simulink model "project"  (R2025a)
settings: Solver=VariableStepAuto  StartTime=0.0  StopTime=0.5  RelTol=1e-3
libraries: spsSeriesRLCBranchLib x7, spsMosfetLib x4, spsVoltageMeasurementLib x3, slpidlib x2, simulink x2, spsCurrentMeasurementLib x2, spsFirstOrderFilterLib x2, spsACVoltageSourceLib x1, spsDiodeLib x1, spsIGBTLib x1, spsPLLLib x1, spsPVArrayLib x1
settings Model: Creator=RYAN CHAN  LastModifiedBy=sharv
settings DebuggingCC: UnconnectedInputMsg=warning  UnconnectedOutputMsg=warning  UnconnectedLineMsg=warning
settings ModelReferenceCC: EnableRefExpFcnMdlSchedulingChecks=on
settings RTWCC: GPUComputeCapability=3.5  DLArmComputeVersion=19.05

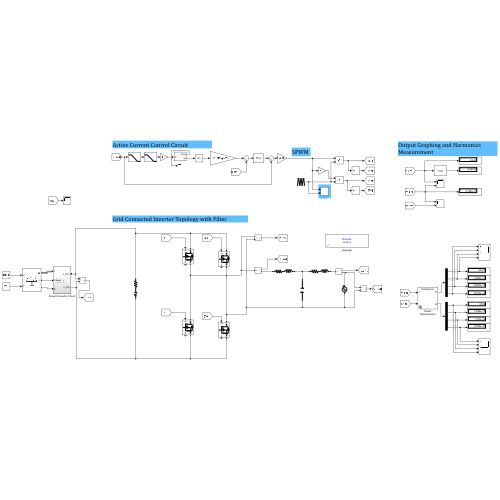
[thumbnail: Simulink's stored preview of the top-level diagram]
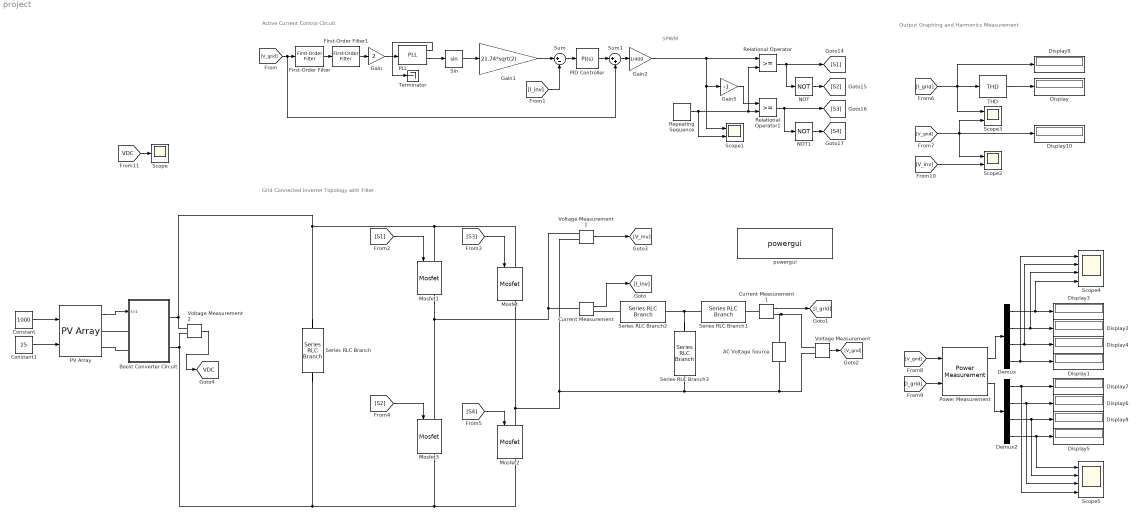
== system project ==
  note: Active Current Control Circuit
  note: Grid Connected Inverter Topology with Filter
  note: SPWM
  note: Output Graphing and Harmonics Measurement
  AC Voltage Source : spsACVoltageSourceLib/AC Voltage Source  Amplitude=230*sqrt(2)  Phase=0  Frequency=50  SampleTime=0  Measurements=None  BusType=swing  Pref=10e3  Qref=0  Qmin=-inf  Qmax=+inf
  Boost Converter Circuit : Subsystem
  Constant : Constant  Value=1000
  Constant1 : Constant  Value=25
  Current Measurement : spsCurrentMeasurementLib/Current Measurement  PhasorSimulation=off  OutputType=Complex  PSBequivalent=0
  Current Measurement1 : spsCurrentMeasurementLib/Current Measurement  PhasorSimulation=off  OutputType=Complex  PSBequivalent=0
  Demux : Demux
  Demux2 : Demux
  Display{,1..10} (11 alike) : Display
  First-Order Filter : spsFirstOrderFilterLib/First-Order Filter  FilterType=Lowpass  Tc=1/(2*pi*50)  Ts=0  Initialize=off  Vac_Init=[0, 0, 60]  Vdc_Init=0  PlotResponse=off  FreqRange="[0,  200,  1]"
  First-Order Filter1 : spsFirstOrderFilterLib/First-Order Filter  FilterType=Lowpass  Tc=1/(2*pi*50)  Ts=0  Initialize=off  Vac_Init=[0, 0, 60]  Vdc_Init=0  PlotResponse=off  FreqRange="[0,  200,  1]"
  Gain : Gain  Gain=2
  Gain1 : Gain  Gain=21.74*sqrt(2)
  Gain2 : Gain  Gain=1/400
  Gain5 : Gain  Gain=-1
  Mosfet{,1..3} (4 alike) : spsMosfetLib/Mosfet  Ron=0.1  Lon=0  Rd=0.01  Vfd=0  IC=0  Rs=1e5  Cs=inf  Measurements=on
  NOT : Logic  Operator=NOT  AllPortsSameDT=off  OutDataTypeStr=boolean
  NOT1 : Logic  Operator=NOT  AllPortsSameDT=off  OutDataTypeStr=boolean
  PID Controller : slpidlib/PID Controller  Controller=PI  Form=Parallel  TimeDomain=Continuous-time  UseExternalTs=off  SampleTime=-1  IntegratorMethod=Forward Euler  FilterMethod=Forward Euler  ControllerParametersSource=internal  P=10.06  I=0.1509  UseKiTs=off  D=0  UseExternalDerivativeSource=off  N=100  UseFilter=on  TunerSelectOption=Transfer Function Based (PID Tuner App)  InitialConditionSource=internal  InitialConditionForIntegrator=0  InitialConditionForFilter=0  DifferentiatorICPrevScaledInput=0  ExternalReset=none  TrackingMode=off  Kt=1  LimitOutput=off  SatLimitsSource=internal  UpperSaturationLimit=inf  LowerSaturationLimit=-inf  LinearizeAsGain=on  AntiWindupMode=none  Kb=1  LimitIntegrator=off  UpperIntegratorSaturationLimit=inf  LowerIntegratorSaturationLimit=-inf  POutMin=[]  POutMax=[]  IOutMin=[]  IOutMax=[]  DOutMin=[]  DOutMax=[]  NOutMin=[]  NOutMax=[]  SumOutMin=[]  SumOutMax=[]  SaturationOutMin=[]  SaturationOutMax=[]  PParamMin=[]  PParamMax=[]  IParamMin=[]  IParamMax=[]  DParamMin=[]  DParamMax=[]  NParamMin=[]  NParamMax=[]  KbParamMin=[]  KbParamMax=[]  KtParamMin=[]  KtParamMax=[]  KbOutMin=[]  KbOutMax=[]  KtOutMin=[]  KtOutMax=[]  IntegratorOutMin=[]  IntegratorOutMax=[]  FilterOutMin=[]  FilterOutMax=[]  SumI1OutMin=[]  SumI1OutMax=[]  SumI2OutMin=[]  SumI2OutMax=[]  SumI3OutMin=[]  SumI3OutMax=[]  SumI4OutMin=[]  SumI4OutMax=[]  SumDOutMin=[]  SumDOutMax=[]  DifferentiatorOutMin=[]  DifferentiatorOutMax=[]  FilterDiffOutCoefMin=[]  FilterDiffOutCoefMax=[]  ReciprocalOutMin=[]  ReciprocalOutMax=[]  SumDenOutMin=[]  SumDenOutMax=[]  SumNumOutMin=[]  SumNumOutMax=[]  DivideOutMin=[]  DivideOutMax=[]  UdiffTsProdOutMin=[]  UdiffTsProdOutMax=[]  NTsProdOutMin=[]  NTsProdOutMax=[]  UintegralTsProdOutMin=[]  UintegralTsProdOutMax=[]  UngainTsProdOutMin=[]  UngainTsProdOutMax=[]  ClampingZeroOutDataTypeStr=Inherit: Inherit via back propagation  ClampingZeroOutMin=[]  ClampingZeroOutMax=[]  FilterDenConstantOutDataTypeStr=Inherit: Inherit via back propagation  FilterDenConstantOutMin=[]  FilterDenConstantOutMax=[]  PCopyOutDataTypeStr=Inherit: Inherit via back propagation  PCopyOutMin=[]  PCopyOutMax=[]  NCopyOutDataTypeStr=Inherit: Inherit via back propagation  NCopyOutMin=[]  NCopyOutMax=[]  IntegratorContinuousStateAttributes=''  IntegratorStateMustResolveToSignalObject=off  IntegratorRTWStateStorageClass=Auto  FilterContinuousStateAttributes=''  FilterStateMustResolveToSignalObject=off  FilterRTWStateStorageClass=Auto  ParallelPVariant=InternalParameters  IdealPVariant=Disabled  IVariant=InternalParameters  DVariant=Disabled  IntegratorVariant=Continuous  SatVariant=Disabled  AWVariant=Passthrough  PCopyVariant=Disabled  TRVariant=Disabled  FdbkBlocksVariant=Forward  IdealPFdbkVariant=Disabled  SatFdbkVariant=Disabled  DerivativeFilterVariant=Disabled  NVariant=Disabled  NCopyVariant=Disabled_SignalSpec  FilterICVariant=Disabled  IntegratorICVariant=InternalICs  ExternalResetVariant=Disabled  TRSumVariant=Passthrough  SumFdbkVariant=Disabled  SumVariant=Sum_PI  TsampFilterVariant=InternalTs  TsampNgainVariant=Passthrough  TsampIntegralVariant=Disabled_SignalSpec  ExternalSaturationOutDataTypeStr=Inherit: Same as second input  DerivativeSourceVariant=Disabled  PreIntVariant=InternalPreInt
  PLL : spsPLLLib/PLL  Fmin=45  Par_Init=[0, 50]  ParK=[180, 3200, 1]  TcD=162e-6  MaxRateChangeFreq=12  FilterCutOffFreq=25  Ts=0  AGC=on
  PV Array : spsPVArrayLib/PV Array  Npar=47  Nser=10  PlotType=array @ 25 deg.C & specified irradiances  S_vec="[ 1000  500  100 ]"  Temp_C_vec="[ 45 25  ]"  ModuleName=User-defined  PlotWhenSelected=off  Pm=213.15  Ncell=60  Voc=36.3  Isc=7.84  Vm=29  Im=7.35  beta_Voc_pc=-0.36099  alpha_Isc_pc=0.102  beta_Voc=-0.13104  alpha_Isc=0.0079968  IL=7.8654  I0=2.9273e-10  nI=0.98119  Rsh=313.0553  Rs=0.39381  RobustModel=off  RobustCellTemperature=313.3991  BAL=on  Tc=1e-6  Tfilter=5e-5
  Power Measurement : eePowerMeasurement/Power Measurement  LabelModeActiveChoice=Continuous  F=50  K=[1 3 5 7]  Ts=0
  Relational Operator : RelationalOperator  OutDataTypeStr=boolean  RndMeth=Simplest  InputSameDT=off
  Relational Operator1 : RelationalOperator  OutDataTypeStr=boolean  RndMeth=Simplest  InputSameDT=off
  Repeating Sequence : simulink/Sources/Repeating Sequence  rep_seq_t=[0 1e-5 2e-5]  rep_seq_y=[-1 1 -1]
  Scope : Scope
      settings: DataLoggingVariableName=ScopeData4
  Scope1 : Scope  NumInputPorts=2
      settings: ActiveDisplayYMinimum=-1.1382  ActiveDisplayYMaximum=0.98886
  Scope2 : Scope  NumInputPorts=2
      settings: ActiveDisplayYMinimum=-406.58639918226481  ActiveDisplayYMaximum=406.58639918226481  DataLoggingVariableName=ScopeData3
  Scope3 : Scope  NumInputPorts=2
      settings: ActiveDisplayYMinimum=-43.30712  ActiveDisplayYMaximum=44.57517  DataLoggingVariableName=ScopeData2
  Scope4 : Scope  NumInputPorts=4
      settings: ActiveDisplayYMinimum=-27.85377883509021  ActiveDisplayYMaximum=31.806771928915644
  Scope5 : Scope  NumInputPorts=4
      settings: ActiveDisplayYMinimum=-12.72391  ActiveDisplayYMaximum=12.80046  DataLoggingVariableName=ScopeData2
  Series RLC Branch : spsSeriesRLCBranchLib/Series RLC Branch  LConnTagsString=__new0  RConnTagsString=__new0  BranchType=RC  Resistance=32  Inductance=1e-3  SetiL0=off  InitialCurrent=0  Capacitance=1e-6  Setx0=off  InitialVoltage=0  Measurements=None
  Series RLC Branch1 : spsSeriesRLCBranchLib/Series RLC Branch  LConnTagsString=__new0  RConnTagsString=__new0  BranchType=RL  Resistance=15e-3  Inductance=1.74e-3  SetiL0=off  InitialCurrent=0  Capacitance=1e-6  Setx0=off  InitialVoltage=0  Measurements=None
  Series RLC Branch2 : spsSeriesRLCBranchLib/Series RLC Branch  LConnTagsString=__new0  RConnTagsString=__new0  BranchType=RL  Resistance=15e-3  Inductance=1.63e-3  SetiL0=off  InitialCurrent=0  Capacitance=1e-6  Setx0=off  InitialVoltage=0  Measurements=None
  Series RLC Branch3 : spsSeriesRLCBranchLib/Series RLC Branch  LConnTagsString=__new0  RConnTagsString=__new0  BranchType=C  Resistance=1e-3  Inductance=1e-3  SetiL0=off  InitialCurrent=0  Capacitance=15e-6  Setx0=off  InitialVoltage=0  Measurements=None
  Sin : Trigonometry
  Sum : Sum  Inputs=|+-
  Sum1 : Sum  Inputs=|++
  THD : spsTHDLib/THD  Freq=50  Ts=0
  Terminator : Terminator
  Voltage Measurement : spsVoltageMeasurementLib/Voltage Measurement  PhasorSimulation=off  OutputType=Complex  PSBequivalent=0
  Voltage Measurement1 : spsVoltageMeasurementLib/Voltage Measurement  PhasorSimulation=off  OutputType=Complex  PSBequivalent=0
  Voltage Measurement2 : spsVoltageMeasurementLib/Voltage Measurement  PhasorSimulation=off  OutputType=Complex  PSBequivalent=0
  powergui : spspowerguiLib/powergui  Priority=1  SimulationMode=Discrete  SampleTime=1e-6  frequency=60  Iterations=50  frequencyindice=50  Pbase=100e6  ErrMax=1e-4  UnitsV=kV  UnitsW=MW  buscounter=0  FunctionMessages=off  echomessages=off  EnableUseOfTLC=off  CurrentSourceSwitches=off  DisableSnubberDevices=off  DisableRonSwitches=off  DisableVfSwitches=off  DisplayEquations=off  AutomaticDiscreteSolvers=off  SolverType=Tustin/Backward Euler (TBE)  Interpol=off  ExternalGateDelay=off  methode=off  Ts=100  x0status=blocks  SPID=on  SwTol=0  HookPort=off  NonlinearTolerance=1e-4  nMaxIteration=100  ContinueOnMaxIteration=off  RestoreLinks=warning  ResistiveCurrentMeasurement=off  Frange=[0:2:500]  Ylog=off  Xlog=on  ShowGrid=off  save=off  variable=ZData  structure=0  ZoomFFT=off  StartTime=0.0  cycles=1  DisplayStyle=1  fundamental=60  FreqAxis=off  MaxFrequency=1000  frequencyindicesteady=1  RmsSteady=1  display=off
  tag scope: VDC=global
  wires:
  [V_grid] -> Sum1/2, First-Order Filter/1
  First-Order Filter/1 -> First-Order Filter1/1
  First-Order Filter1/1 -> Gain/1
  Sin/1 -> Gain1/1
  Gain1/1 -> Sum/1
  Sum/1 -> PID Controller/1
  [I_inv] -> Sum/2
  PID Controller/1 -> Sum1/1
  Sum1/1 -> Gain2/1
  Gain2/1 -> Relational Operator/1, Scope1/1, Gain5/1
  Relational Operator1/1 -> NOT1/1, [S3]
  NOT1/1 -> [S4]
  NOT/1 -> [S2]
  Gain5/1 -> Relational Operator1/1
  Repeating Sequence/1 -> Scope1/2, Relational Operator1/2, Relational Operator/2
  Relational Operator/1 -> NOT/1, [S1]
  Current Measurement1/1 -> [I_grid]
  [S3] -> Mosfet/1
  Current Measurement/1 -> [I_inv]
  [S1] -> Mosfet1/1
  Voltage Measurement/1 -> [V_grid]
  [S2] -> Mosfet3/1
  [S4] -> Mosfet2/1
  Gain/1 -> PLL/1
  PLL/2 -> Sin/1
  PLL/1 -> Terminator/1
  [I_grid] -> Display9/1, THD/1, Scope3/1
  [V_grid] -> Scope2/1, Display10/1, Scope3/2
  THD/1 -> Display/1
  [I_grid] -> Power Measurement/2
  [V_grid] -> Power Measurement/1
  Power Measurement/1 -> Demux/1
  Demux/3 -> Scope4/2, Display4/1
  Demux/1 -> Scope4/4, Display3/1
  Demux/4 -> Display1/1, Scope4/1
  Demux/2 -> Scope4/3, Display2/1
  Demux2/2 -> Scope5/3, Display6/1
  Demux2/4 -> Scope5/1, Display5/1
  Demux2/1 -> Scope5/4, Display7/1
  Demux2/3 -> Display8/1, Scope5/2
  Power Measurement/2 -> Demux2/1
  Voltage Measurement1/1 -> [V_inv]
  [V_inv] -> Scope2/2
  PV Array/1 -> Boost Converter Circuit/1(In1)
  Constant1/1 -> PV Array/2
  Voltage Measurement2/1 -> [VDC]
  Constant/1 -> PV Array/1
  [VDC] -> Scope/1
  connections:
  Voltage Measurement/LConn2 -- AC Voltage Source/LConn1 -- Series RLC Branch3/RConn1 -- Voltage Measurement1/LConn2 -- Mosfet2/LConn1 -- Mosfet/RConn1
  Voltage Measurement/LConn1 -- Current Measurement1/RConn1 -- AC Voltage Source/RConn1
  Boost Converter Circuit/RConn2 -- Mosfet2/RConn1 -- Mosfet3/RConn1 -- Series RLC Branch/RConn1 -- Voltage Measurement2/LConn2
  Current Measurement/LConn1 -- Voltage Measurement1/LConn1 -- Mosfet3/LConn1 -- Mosfet1/RConn1
  Boost Converter Circuit/RConn1 -- Voltage Measurement2/LConn1 -- Mosfet1/LConn1 -- Mosfet/LConn1 -- Series RLC Branch/LConn1
  Series RLC Branch2/RConn1 -- Series RLC Branch1/LConn1 -- Series RLC Branch3/LConn1
  Current Measurement1/LConn1 -- Series RLC Branch1/RConn1
  Series RLC Branch2/LConn1 -- Current Measurement/RConn1
  Boost Converter Circuit/LConn1 -- PV Array/RConn1
  Boost Converter Circuit/LConn2 -- PV Array/RConn2

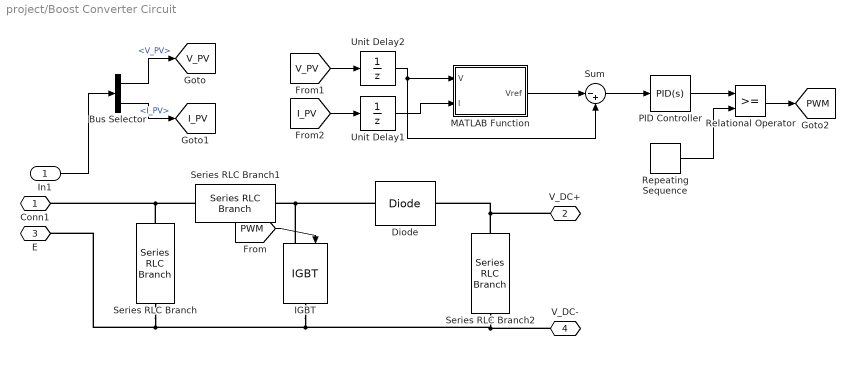
== system project/Boost Converter Circuit ==
  In1 : Inport
  Bus Selector : BusSelector  OutputSignals=V_PV,I_PV
  Diode : spsDiodeLib/Diode  Ron=0.001  Lon=0  Vf=0.8  IC=0  UseSnubber=0  Rs=500  Cs=250e-9  Measurements=off
  IGBT : spsIGBTLib/IGBT  Ron=0.001  Lon=0  Vf=1  Tf=1e-6  Tt=2e-6  IC=0  Rs=1e5  Cs=inf  Measurements=off
  MATLAB Function : MATLAB Function  TreatAsAtomicUnit=on
  PID Controller : slpidlib/PID Controller  Controller=PID  Form=Parallel  TimeDomain=Continuous-time  UseExternalTs=off  SampleTime=-1  IntegratorMethod=Forward Euler  FilterMethod=Forward Euler  ControllerParametersSource=internal  P=0.005  I=0.001  UseKiTs=off  D=0  UseExternalDerivativeSource=off  N=100  UseFilter=on  TunerSelectOption=Transfer Function Based (PID Tuner App)  InitialConditionSource=internal  InitialConditionForIntegrator=0  InitialConditionForFilter=0  DifferentiatorICPrevScaledInput=0  ExternalReset=none  TrackingMode=off  Kt=1  LimitOutput=on  SatLimitsSource=internal  UpperSaturationLimit=0.95  LowerSaturationLimit=0  LinearizeAsGain=on  AntiWindupMode=none  Kb=1  LimitIntegrator=off  UpperIntegratorSaturationLimit=inf  LowerIntegratorSaturationLimit=-inf  POutMin=[]  POutMax=[]  IOutMin=[]  IOutMax=[]  DOutMin=[]  DOutMax=[]  NOutMin=[]  NOutMax=[]  SumOutMin=[]  SumOutMax=[]  SaturationOutMin=[]  SaturationOutMax=[]  PParamMin=[]  PParamMax=[]  IParamMin=[]  IParamMax=[]  DParamMin=[]  DParamMax=[]  NParamMin=[]  NParamMax=[]  KbParamMin=[]  KbParamMax=[]  KtParamMin=[]  KtParamMax=[]  KbOutMin=[]  KbOutMax=[]  KtOutMin=[]  KtOutMax=[]  IntegratorOutMin=[]  IntegratorOutMax=[]  FilterOutMin=[]  FilterOutMax=[]  SumI1OutMin=[]  SumI1OutMax=[]  SumI2OutMin=[]  SumI2OutMax=[]  SumI3OutMin=[]  SumI3OutMax=[]  SumI4OutMin=[]  SumI4OutMax=[]  SumDOutMin=[]  SumDOutMax=[]  DifferentiatorOutMin=[]  DifferentiatorOutMax=[]  FilterDiffOutCoefMin=[]  FilterDiffOutCoefMax=[]  ReciprocalOutMin=[]  ReciprocalOutMax=[]  SumDenOutMin=[]  SumDenOutMax=[]  SumNumOutMin=[]  SumNumOutMax=[]  DivideOutMin=[]  DivideOutMax=[]  UdiffTsProdOutMin=[]  UdiffTsProdOutMax=[]  NTsProdOutMin=[]  NTsProdOutMax=[]  UintegralTsProdOutMin=[]  UintegralTsProdOutMax=[]  UngainTsProdOutMin=[]  UngainTsProdOutMax=[]  ClampingZeroOutDataTypeStr=Inherit: Inherit via back propagation  ClampingZeroOutMin=[]  ClampingZeroOutMax=[]  FilterDenConstantOutDataTypeStr=Inherit: Inherit via back propagation  FilterDenConstantOutMin=[]  FilterDenConstantOutMax=[]  PCopyOutDataTypeStr=Inherit: Inherit via back propagation  PCopyOutMin=[]  PCopyOutMax=[]  NCopyOutDataTypeStr=Inherit: Inherit via back propagation  NCopyOutMin=[]  NCopyOutMax=[]  IntegratorContinuousStateAttributes=''  IntegratorStateMustResolveToSignalObject=off  IntegratorRTWStateStorageClass=Auto  FilterContinuousStateAttributes=''  FilterStateMustResolveToSignalObject=off  FilterRTWStateStorageClass=Auto  ParallelPVariant=InternalParameters  IdealPVariant=Disabled  IVariant=InternalParameters  DVariant=InternalParameters  IntegratorVariant=Continuous  SatVariant=Enabled  AWVariant=Passthrough  PCopyVariant=Disabled  TRVariant=Disabled  FdbkBlocksVariant=Forward  IdealPFdbkVariant=Disabled  SatFdbkVariant=Disabled  DerivativeFilterVariant=ContFilter  NVariant=InternalParameters  NCopyVariant=Disabled  FilterICVariant=InternalICsFilter  IntegratorICVariant=InternalICs  ExternalResetVariant=Disabled  TRSumVariant=Passthrough  SumFdbkVariant=Disabled  SumVariant=Sum_PID  TsampFilterVariant=InternalTs  TsampNgainVariant=Passthrough  TsampIntegralVariant=Disabled_SignalSpec  ExternalSaturationOutDataTypeStr=Inherit: Same as second input  DerivativeSourceVariant=ErrorSignal  PreIntVariant=InternalPreInt
  Relational Operator : RelationalOperator  OutDataTypeStr=boolean  RndMeth=Simplest  InputSameDT=off
  Repeating Sequence : simulink/Sources/Repeating Sequence  rep_seq_t=[0 0.0002]  rep_seq_y=[0 1]
  Series RLC Branch : spsSeriesRLCBranchLib/Series RLC Branch  LConnTagsString=__new0  RConnTagsString=__new0  BranchType=RC  Resistance=1e-3  Inductance=1e-3  SetiL0=off  InitialCurrent=0  Capacitance=1000e-6  Setx0=off  InitialVoltage=0  Measurements=None
  Series RLC Branch1 : spsSeriesRLCBranchLib/Series RLC Branch  LConnTagsString=__new0  RConnTagsString=__new0  BranchType=L  Resistance=0.0001  Inductance=1.45e-3  SetiL0=off  InitialCurrent=0  Capacitance=1000e-6  Setx0=off  InitialVoltage=0  Measurements=None
  Series RLC Branch2 : spsSeriesRLCBranchLib/Series RLC Branch  LConnTagsString=__new0  RConnTagsString=__new0  BranchType=C  Resistance=0.0001  Inductance=1.45e-3  SetiL0=off  InitialCurrent=0  Capacitance=3227e-6  Setx0=off  InitialVoltage=0  Measurements=None
  Sum : Sum  Inputs=|-+
  Unit Delay1 : UnitDelay  SampleTime=1e-4  HasFrameUpgradeWarning=on
  Unit Delay2 : UnitDelay  SampleTime=1e-4  HasFrameUpgradeWarning=on
  Conn1 : PMIOPort  Side=Left
  V_DC+ : PMIOPort  Port=2  Side=Right
  E : PMIOPort  Port=3  Side=Left
  V_DC- : PMIOPort  Port=4  Side=Right
  tag scope: I_PV=global, PWM=global, V_PV=global
  wires:
  Bus Selector/2 -> [I_PV]  "<I_PV>"
  Sum/1 -> PID Controller/1
  [V_PV] -> Unit Delay2/1
  Repeating Sequence/1 -> Relational Operator/2
  Unit Delay2/1 -> MATLAB Function/1(V), Sum/2
  [PWM] -> IGBT/1
  MATLAB Function/1(Vref) -> Sum/1
  PID Controller/1 -> Relational Operator/1
  [I_PV] -> Unit Delay1/1
  Unit Delay1/1 -> MATLAB Function/2(I)
  Bus Selector/1 -> [V_PV]  "<V_PV>"
  Relational Operator/1 -> [PWM]
  In1/1 -> Bus Selector/1
  connections:
  Series RLC Branch1/LConn1 -- Series RLC Branch/LConn1 -- Conn1/RConn1
  E/RConn1 -- Series RLC Branch/RConn1 -- IGBT/RConn1 -- V_DC-/RConn1 -- Series RLC Branch2/RConn1
  Series RLC Branch1/RConn1 -- IGBT/LConn1 -- Diode/LConn1
  Diode/RConn1 -- Series RLC Branch2/LConn1 -- V_DC+/RConn1

== matlab function project/Boost Converter Circuit/MATLAB Function ==
  data: Vref output; V input; I input
function Vref = RefGen(V, I)

VrefMax = 363;
Vrefmin = 0;
Vrefinit = 300;
deltaVref = 1;
persistent Vold Pold Vrefold;

dataType = 'double';

if isempty(Vold)
    Vold = 0;
    Pold = 0;
    Vrefold = Vrefinit;
end

P = V * I;
dV = V - Vold;
dP = P - Pold;

if dP ~= 0
    if dP < 0
        if dV<0
            Vref = Vrefold + deltaVref;
        else
            Vref = Vrefold - deltaVref;
        end
    else
        if dV < 0
            Vref = Vrefold - deltaVref;
        else
            Vref = Vrefold + deltaVref;
        end
    end

else Vref = Vrefold;
end

if Vref >= VrefMax | Vref <= Vrefmin
    Vref = Vrefold;
end

Vrefold = Vref;
Vold = V;
Pold=P;
